simulink model "RL_SMC_Training_Env"  (R2024b)
settings: Solver=VariableStepAuto  StartTime=0.0  StopTime=60  RelTol=1e-3
values from neighbouring files (symbols this model uses):
  D = [0; 0]    [K_vector_2.m]
undefined symbols (not defined in the file or in its folder): ref_seed
libraries: simulink x2, rllib x2
(part 2 of 2)

== matlab function RL_SMC_Training_Env/MATLAB Function1 ==
  data: u1 input; C2 output; u2 input; u3 input; u4 input; C4 output; Eta output; Phi output
function [C2, C4, Eta, Phi] = scale_actions(u1, u2, u3, u4)
    % =====================================================================
    % scale_actions.m
    % Converts the normalized [-1, 1] AI outputs into safe physical tuning 
    % boundaries for the Sliding Mode Controller.
    % =====================================================================

    % --- ENFORCE STRICT DATA TYPES ---
    u_1 = double(u1);
    u_2 = double(u2);
    u_3 = double(u3);
    u_4 = double(u4);

    % --- 1. C2: Speed vs. Overshoot ---
    % Baseline: 20.0 | Ceiling: 25.0 | Safe Range: [15.0 to 25.0]
    % If u1 = 1, C2 = 25. If u1 = -1, C2 = 15.
    C2 = double(20.0 + (5.0 * u_1));

    % --- 2. C4: Damping ---
    % Baseline: 2.0 | Scale: 1.0 | Safe Range: [1.0 to 3.0]
    C4 = double(2.0 + (1.0 * u_2));

    % --- 3. Eta: Reaching Law (Steady-State Error) ---
    % Center: 100.0 | Scale: 50.0 | Safe Range: [50.0 to 150.0]
    Eta = double(100.0 + (50.0 * u_3));

    % --- 4. Phi: Boundary Layer (Chatter Killer) ---
    % Center: 0.100 | Scale: 0.070 | Safe Range: [0.030 to 0.170]
    % Ensures Phi never drops below the 0.027 chatter threshold.
    Phi = double(0.100 + (0.070 * u_4));
end

== matlab function RL_SMC_Training_Env/Reward2 ==
  data: x1 input; x2 input; x2_ref input; u input; time_since_change input; v1 input; v2 input; reward output; next_u_prev output; u_prev input
function [reward, next_u_prev] = calc_reward(x1, x2, x2_ref, u, time_since_change, v1, v2, u_prev)

% =========================================================================
% calc_reward.m — Phase 1: 50Hz Bounded Slalom
% Focus: Smooth tracking, scaled continuous rewards.
% =========================================================================

% --- ENFORCE STRICT DATA TYPES ---
    reward       = double(0.2);           % Scaled base survival
    next_u_prev  = double(u);             
    x2_error     = double(abs(x2_ref - x2));
    delta_u      = double(abs(u - u_prev));
    x1_abs       = double(abs(x1));
    delta_u_sum  = double(sum(abs(u - u_prev)));

% --- 1. TRACKING (RISE TIME AGGRESSION) ---
    reward = double(reward - (4.0 * x2_error^2));

% --- 2. FORGIVING PARACHUTE (50mm warning zone) ---
    if (x2_error < 0.050) && (abs(v2) > 0.10)
        reward = double(reward - (1.0 * abs(v2)));
    end

% --- 3. TARGET LOCK BONUS ---
    if x2_error < 0.010
        reward = double(reward + 0.6);    % inside 10mm 
    elseif x2_error < 0.030
        reward = double(reward + 0.3);    % inside 30mm (Matches Settle Boundary)
    end

% --- 4. CONTINUOUS PROGRESS BONUS ---
    progress_bonus = double(0.2 * exp(-5.0 * x2_error^2));
    reward = double(reward + progress_bonus);

% --- 5. CHATTER REDUCTION (SMOOTH THE SMC) ---
    % The max possible sum is 8.0. If the AI moves its joysticks more than 
    % a combined 0.2 (10% total shift) in a single 0.02s frame, penalize it.
    if delta_u_sum > 0.2
        reward = double(reward - (0.05 * delta_u_sum));
    end
    
% --- 6. X1 SOFT BARRIER & CENTERING ---
    if x1_abs > 0.30
        x1_margin1 = double(x1_abs - 0.30);
        reward = double(reward - (1.6 * x1_margin1^2));
    end
    x1_centre_bonus = double(0.06 * exp(-10.0 * x1^2));
    reward = double(reward + x1_centre_bonus);

% --- 7. TERMINAL PENALTY ---
    if x1_abs > 0.65
        reward = double(reward - 200.0);
    end

% --- 8. PER-STEP HARD FLOOR ---
    reward = double(max(reward, -10.0));

end

== matlab function RL_SMC_Training_Env/IsDone2 ==
  data: x1 input; is_done output; x2 input; x2_ref input; next_timer_03 output; timer_03 input; time_since_change input; current_step_size input; x2_ref_prev input; next_time_since_change output; next_step_size output; next_ref_prev output
function [is_done, next_timer_03, next_time_since_change, next_step_size, next_ref_prev] = check_safety(x1, x2, x2_ref, timer_03, time_since_change, current_step_size, x2_ref_prev)

% =========================================================================
% check_safety.m — Phase 1: 50Hz Bounded Slalom
% Focus: 2.5s Settle-Time & Hardware Protection
% =========================================================================

% --- ENFORCE STRICT DATA TYPES ---
    is_done                = double(0);
    next_timer_03          = double(timer_03);
    next_time_since_change = double(time_since_change);
    next_step_size         = double(current_step_size);
    next_ref_prev          = double(x2_ref_prev);
    
    dt       = double(0.02); % 50Hz AI clock 
    x2_error = double(x2_ref - x2);

% --- 1. REFERENCE CHANGE DETECTION ---
    if abs(x2_ref - x2_ref_prev) > 0.001
        next_time_since_change = double(0.0);
        next_step_size         = double(abs(x2_ref - x2_ref_prev));
    else
        next_time_since_change = double(time_since_change + dt);
    end
    next_ref_prev = double(x2_ref);

% --- 2. DEATH A: Hardware Limit (x1 wall) ---
    if abs(x1) > 0.65
        is_done = double(1);
    end

% --- 3. DEATH B: Total Loss of Control ---
    if abs(x2_error) > 0.5
        next_timer_03 = double(timer_03 + dt);
    else
        next_timer_03 = double(0.0);
    end
    
    if next_timer_03 > 3.0
        is_done = double(1);
    end

% --- 4. DEATH C: The Slalom Settle-Time ---
% Because the jump happens every 3.0s, give it 2.5s to settle.
    allowed_settle_time = double(2.5);
    error_band          = double(0.030); % Forgiving 30mm boundary
    
    if (next_time_since_change > allowed_settle_time) && (abs(x2_error) > error_band)
        is_done = double(1);
    end

end
